simulink model "Driver_test"  (R2025b)
settings: Solver=FixedStepDiscrete  StartTime=0.0  StopTime=69.2  FixedStep=1e-4  RelTol=1e-3
PreLoadFcn:
  | controller_params
InitFcn:
  | controller_params
values from neighbouring files (symbols this model uses):
  vBias = 0.3    [analyse_driver.m]
undefined symbols (not defined in the file or in its folder): Ao, Bo, DiscIntNeverNeededParam, K, Ke, Pull, tExc, Ts, up, vMax
libraries: speedgoatlib_IO183 x3, simulink x1
settings Model: SimulationMode=external  Creator=rafaeltavares  LastModifiedBy=havard
settings SolverCC: ConcurrentTasks=on  AlgebraicLoopSolver=TrustRegion  PositivePriorityOrder=on  InsertRTBMode=Never (minimum delay)
settings DataIOCC: SaveFormat=StructureWithTime  ReturnWorkspaceOutputs=off
settings OptimizationCC: BlockReduction=off  OptimizeBlockIOStorage=off  BufferReuse=off  GlobalBufferReuse=off  ExpressionFolding=off  LocalBlockOutputs=off  OptimizeDataStoreBuffers=off  BusAssignmentInplaceUpdate=off
settings DebuggingCC: TasksWithSamePriorityMsg=none  UnconnectedInputMsg=warning  UnconnectedOutputMsg=warning  UnconnectedLineMsg=warning  UnderSpecifiedDimensionMsg=warning  ArithmeticOperatorsInVariantConditions=warning
settings HardwareCC: ProdBitPerLong=64.0  ProdLongLongMode=on  ProdHWDeviceType=Intel->x86-64 (Linux 64)
settings ModelReferenceCC: EnableRefExpFcnMdlSchedulingChecks=on
settings SFSimCC: CustomCodeUndefinedFunction=UseInterfaceOnly
settings RTWCC: SystemTargetFile=speedgoat.tlc  TemplateMakefile=slrealtime_default_tmf  Toolchain=Simulink Real-Time Toolchain  BuildConfiguration=Faster Runs  CodeExecutionProfiling=on  TargetLang=C++  GPUComputeCapability=3.5  DLArmComputeVersion=19.05  Description=Speedgoat Real-Time Target Machine
settings SimulinkRealTimeTargetCC: SLRTFileLogMaxRuns=1.0  ExtModeMaxTrigDuration=10.0  ExtModeStaticAllocSize=1000000.0  ExtModeTransport=0.0  MultiwordLength=2048.0  DynamicStringBufferSize=256.0  PreserveMATLABNamespacesInGeneratedCode=on  SubcomponentCodeInterfacePackaging=Reusable function  InstructionSetFMA=off  LogToMDFFile=off

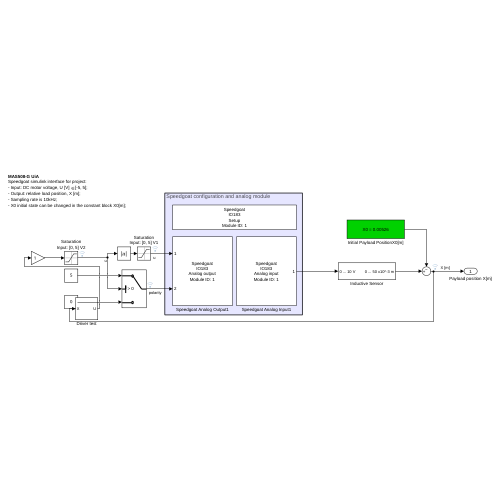
[thumbnail: Simulink's stored preview of the top-level diagram]
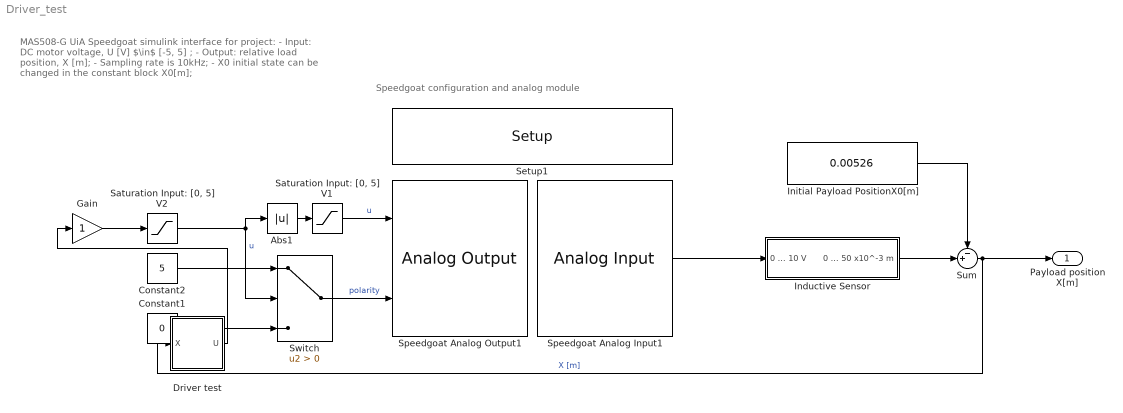
== system Driver_test ==
  note: MAS508-G UiA
      | Speedgoat simulink interface for project:
      | - Input: DC motor voltage, U [V] $\in$ [-5, 5] ;
      | - Output: relative load position, X [m];
      | - Sampling rate is 10kHz;
      | - X0 initial state can be changed in the constant block X0[m];
  note: Speedgoat configuration and analog module
  Abs1 : Abs  SaturateOnIntegerOverflow=off
  Constant1 : Constant  Value=0
  Constant2 : Constant  Value=5
  Driver test : Subsystem
  Gain : Gain
  "Inductive Sensor " : Subsystem
  "Initial Payload PositionX0[m] " : Constant  Value=0.00526
      mask Display:
      | set_param(gcb,'BackgroundColor','green');
      | fprintf('X0 = %s', get_param(gcb,'Value'))
  "Saturation Input: [0, 5] V1" : Saturate  UpperLimit=5  LowerLimit=0
  "Saturation Input: [0, 5] V2" : Saturate  UpperLimit=5  LowerLimit=-5
  Setup1 : speedgoatlib_IO183/Setup  parModuleId=1  parPciSlot=-1  parDaSimult=on  parAdCoupling=Single Ended  parAdRange=0..10V  parAdChannelLow=1  parAdChannelHigh=1  parDaChannels=[1 2]  parDaRange=0..5V  parDaInit=[0 5 0 0]  parDaReset=1  parDoChannels=[1:8]  parDoInit=[0]  parDoReset=[1]  parDiChannels=[9:16]  parIOPullReferenceFront=Pull-up (3.3V)  parIOPullReferenceRear=Pull-up (3.3V)
      settings: SourceProductName=IO183
  Speedgoat Analog Input1 : speedgoatlib_IO183/Analog Input  Priority=0  parModuleId=1  parSampTime=-1  parPciSlot=-1  parAdChannelLow=1  parAdChannelHigh=1
      settings: SourceProductName=IO183
  Speedgoat Analog Output1 : speedgoatlib_IO183/Analog Output  parModuleId=1  parSampTime=-1  parDaSimult=on  parPciSlot=-1  parDaChannels=[1 2]  parDaInit=[0 5 0 0]  parDaReset=[1 1 1 1]
      settings: SourceProductName=IO183
  Sum : Sum  Inputs=-+|
  Switch : Switch  Criteria=u2 > Threshold  SaturateOnIntegerOverflow=off  InputSameDT=off
  Payload position X[m] : Outport
  wires:
  "Inductive Sensor "/1(0 ... 50 x10^-3 m) -> Sum/2
  "Initial Payload PositionX0[m] "/1 -> Sum/1
  "Saturation Input: [0, 5] V1"/1 -> Speedgoat Analog Output1/1  "u"
  Constant2/1 -> Switch/1
  Speedgoat Analog Input1/1 -> "Inductive Sensor "/1(0 ... 10 V)
  Abs1/1 -> "Saturation Input: [0, 5] V1"/1
  Switch/1 -> Speedgoat Analog Output1/2  "polarity"
  Constant1/1 -> Switch/3
  Gain/1 -> "Saturation Input: [0, 5] V2"/1
  "Saturation Input: [0, 5] V2"/1 -> Switch/2, Abs1/1  "u"
  Sum/1 -> Payload position X[m]/1, Driver test/1(X)  "X [m]"
  Driver test/1(U) -> Gain/1

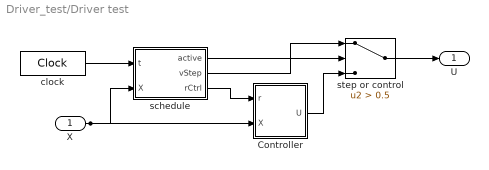
== system Driver_test/Driver test ==
  X : Inport
  Controller : Subsystem
  clock : DigitalClock  SampleTime=Ts
  schedule : MATLAB Function  TreatAsAtomicUnit=on
  step or control : Switch  Criteria=u2 > Threshold  Threshold=0.5  SaturateOnIntegerOverflow=off  InputSameDT=off
  U : Outport
  wires:
  schedule/3(rCtrl) -> Controller/1(r)
  Controller/1(U) -> step or control/3
  schedule/2(vStep) -> step or control/1
  schedule/1(active) -> step or control/2
  step or control/1 -> U/1
  X/1 -> schedule/2(X), Controller/2(X)
  clock/1 -> schedule/1(t)

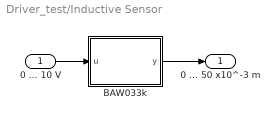
== system Driver_test/Inductive Sensor  ==
  0 ... 10 V : Inport
  BAW033k : MATLAB Function  TreatAsAtomicUnit=on
  0 ... 50 x10^-3 m : Outport  VectorParamsAs1DForOutWhenUnconnected=off
  wires:
  BAW033k/1(y) -> 0 ... 50 x10^-3 m/1
  0 ... 10 V/1 -> BAW033k/1(u)

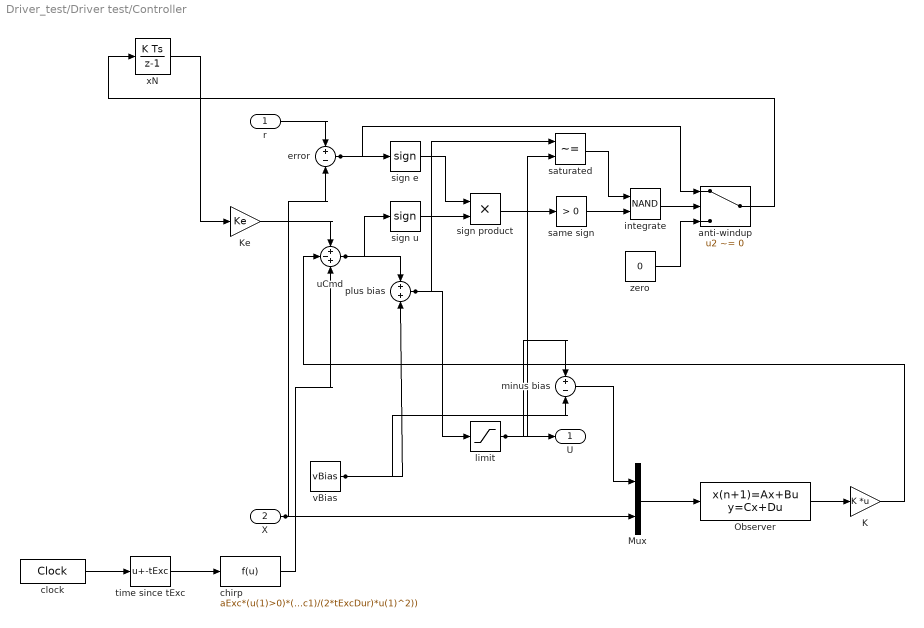
== system Driver_test/Driver test/Controller ==
  r : Inport
  X : Inport  Port=2
  K : Gain  Gain=K  Multiplication=Matrix(K*u)
  Ke : Gain  Gain=Ke
  Mux : Mux  Inputs=2
  Observer : DiscreteStateSpace  A=Ao  B=Bo  C=eye(5)  D=zeros(5, 2)  SampleTime=Ts
  anti-windup : Switch  Criteria=u2 ~= 0  SaturateOnIntegerOverflow=off  InputSameDT=off
  chirp : Fcn  Expr=aExc*(u(1)>0)*(u(1)<tExcDur)*sin(2*pi*(fExc1*u(1) + (fExc2-fExc1)/(2*tExcDur)*u(1)^2))
  clock : DigitalClock  SampleTime=Ts
  error : Sum  Inputs=+-
  integrate : Logic  Operator=NAND  AllPortsSameDT=off  OutDataTypeStr=boolean
  limit : Saturate  UpperLimit=vMax  LowerLimit=-vMax
  minus bias : Sum  Inputs=+-
  plus bias : Sum
  same sign : simulink/Logic and Bit Operations/Compare To Constant  relop=>  const=0  OutDataTypeStr=boolean
  saturated : RelationalOperator  Operator=~=  OutDataTypeStr=boolean  RndMeth=Simplest  InputSameDT=off
  sign e : Signum
  sign product : Product
  sign u : Signum
  time since tExc : Bias  Bias=-tExc  SaturateOnIntegerOverflow=off
  uCmd : Sum  Inputs=+-+
  vBias : Constant  Value=vBias
  xN : DiscreteIntegrator  SampleTime=Ts  ICPrevOutput=DiscIntNeverNeededParam  ICPrevScaledInput=DiscIntNeverNeededParam
  zero : Constant  Value=0
  U : Outport
  wires:
  plus bias/1 -> saturated/1, limit/1
  sign u/1 -> sign product/2
  xN/1 -> Ke/1
  Mux/1 -> Observer/1
  sign e/1 -> sign product/1
  r/1 -> error/1
  uCmd/1 -> plus bias/1, sign u/1
  saturated/1 -> integrate/1
  vBias/1 -> minus bias/2, plus bias/2
  error/1 -> anti-windup/1, sign e/1
  zero/1 -> anti-windup/3
  chirp/1 -> uCmd/3
  time since tExc/1 -> chirp/1
  X/1 -> Mux/2, error/2
  Ke/1 -> uCmd/1
  clock/1 -> time since tExc/1
  sign product/1 -> same sign/1
  limit/1 -> minus bias/1, U/1, saturated/2
  same sign/1 -> integrate/2
  anti-windup/1 -> xN/1
  minus bias/1 -> Mux/1
  integrate/1 -> anti-windup/2
  Observer/1 -> K/1
  K/1 -> uCmd/2

== matlab function Driver_test/Driver test/schedule ==
  data: t input; active output; X input; vStep output; rCtrl output
function [active, vStep, rCtrl] = schedule(t, X)
[active, vStep, rCtrl] = driver_schedule(t, X);

== matlab function Driver_test/Inductive Sensor /BAW033k ==
  data: u input; y output
function y = fcn(u)
% Input: 0 ... 10 V
% Output: 0 ... 40 mm
y =(40*10^-3/10)*u; %Output in SI [m]
